simulink model "MMC_phase_hackathon_circuit3_HAAS_20260216"  (R2024b)
settings: Solver=FixedStepDiscrete  StartTime=t_init_sim  StopTime=sim_time  FixedStep=Ts  RelTol=1e-3
values from neighbouring files (symbols this model uses):
  a = 1    [param_phase_circuit3_20260216.m]
  C1low1_active = 1    [script_MMC_phase_circuit3_twist_20260216.m]
  C2low1_active = 1    [script_MMC_phase_circuit3_twist_20260216.m]
  C_bus = 4400e-6    (= 0.0044)    [param_phase_circuit3_20260216.m]
  C_M_extra = C_m-twist_high_side_C    [param_phase_circuit3_20260216.m]
  duty_cycle = 0.95    [script_MMC_phase_circuit3_twist_20260216.m]
  f0 = 50    [param_phase_circuit3_20260216.m]
  feeder_current_lower_rate_limit = -10    [script_MMC_phase_circuit3_twist_20260216.m]    (also in twist_parameters.m = -500)
  feeder_current_tab = [0.328 0.217 0.162 0.132 0.109 0.094 0.083 0.075 0.068 0.062 0.058 0.054 ... (42 elements, 14x3)]    [feeder_current.mat]
  feeder_current_upper_rate_limit = 0.386/(20e-3)    (= 19.3)    [twist_parameters.m]
  is6VExternallySupplied = true    [script_MMC_phase_circuit3_twist_20260216.m]
  isFeederJumperOpen = true    [script_MMC_phase_circuit3_twist_20260216.m]
  L_arm = 60e-3    (= 0.06)    [param_phase_circuit3_20260216.m]
  m = 1    [param_phase_circuit3_20260216.m]
  N = 5    [param_phase_circuit3_20260216.m]
  power_losses = false    [script_MMC_phase_circuit3_twist_20260216.m]
  R = 15    [param_phase_circuit3_20260216.m]
  source_V = 0    [script_MMC_phase_circuit3_twist_20260216.m]
  time_charge = 0.1    [script_MMC_phase_circuit3_twist_20260216.m]
  time_decharge = 0.6    [script_MMC_phase_circuit3_twist_20260216.m]
  Ts = 5e-7    (= 5e-07)    [script_MMC_phase_circuit3_twist_20260216.m]
  twist_data_acquisition_delay = 50e-9    (= 5e-08)    [script_MMC_phase_circuit3_twist_20260216.m]    (also in twist_parameters.m)
  twist_data_sampling_period = 1/twist_freq_data_sampling    (= 5e-05)    [script_MMC_phase_circuit3_twist_20260216.m]    (also in twist_parameters.m)
  twist_dead_time = 200e-9    (= 2e-07)    [twist_parameters.m]
  twist_freq_switching = 200e3    (= 200000)    [twist_parameters.m]
  twist_high_side_adc_R = 1/(1/2e6 + 1/2e6 + 1/(330e3+5.6e3))    (= 251272.836178)    [twist_parameters.m]
  twist_high_side_C = 33e-6*4 + 4.7e-6*12    (= 0.0001884)    [twist_parameters.m]
  twist_high_side_feeder_R = 47e3+4.7e3    (= 51700)    [twist_parameters.m]
  twist_high_side_rC = 0.1    [twist_parameters.m]
  twist_low_side_adc_R = 150e3+470    (= 150470)    [twist_parameters.m]
  twist_low_side_C_ceramic = 3*4.7e-6    (= 1.41e-05)    [twist_parameters.m]
  twist_low_side_C_electrolytic = 47e-6    (= 4.7e-05)    [twist_parameters.m]
  twist_low_side_L = 33e-6    (= 3.3e-05)    [twist_parameters.m]
  twist_low_side_rC = 700e-3    (= 0.7)    [twist_parameters.m]
  twist_low_side_rL = 20e-3    (= 0.02)    [twist_parameters.m]
  twist_R_VCC = (tau_VCC/twist_high_side_C  - twist_high_side_rC)/(1-(tau_VCC/twist_high_side_C - twist_high_side_rC)/R_parallel)    (= 1110.74997822)    [twist_parameters.m]
  VDC = 48    [param_phase_circuit3_20260216.m]
undefined symbols (not defined in the file or in its folder): C_SM, feeder_current, gcbh, sps_rtmsupport, twist_low_side_lC
libraries: spsSeriesRLCBranchLib x133, spsTriangleGeneratorLib x60, spsMosfetLib x60, spsVoltageMeasurementLib x55, spsCurrentMeasurementLib x43, spsControlledCurrentSourceLib x30, spsDiodeLib x22, spsIdealSwitchLib x20, spsControlledVoltageSourceLib x1, spsGroundLib x1, spsMeanLib x1, spspowerguiLib x1
(part 5 of 18)

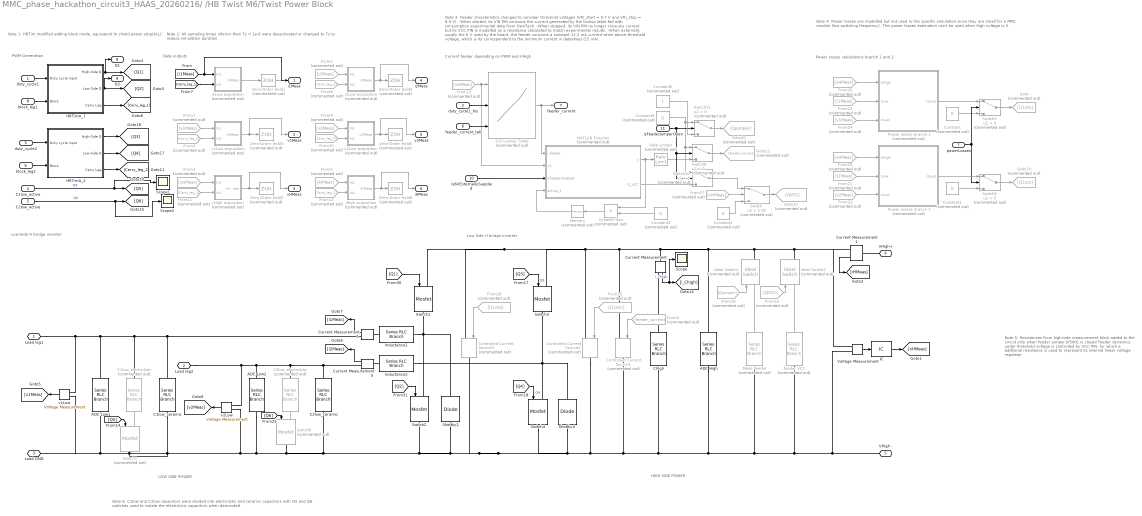
== system MMC_phase_hackathon_circuit3_HAAS_20260216/ /HB Twist M6/Twist Power Block ==
  note: Power losses calculations branch 1 and 2
  note: Current feeder depending on PWM and VHigh
  note: LOW SIDE POWER
  note: Data outputs
  note: PWM Generation
  note: Low-Side H bridge inverter
  note: Low Side H bridge inverter
  note: HIGH SIDE POWER
  note: Note 1:
      | HRTim modified adding block mode, equivalent to shield.power.stop(ALL);
  note: Note 2:
      | All sampling times inferior than Ts = 1e-6 were desactivated or changed to Ts to reduce simulation duration
  note: Note 3:
      | Feeder chracteristics changed to consider threshold voltages (Vth_start = 9.7 V and Vth_stop = 8.9 V).
      | -When started, its VIN PIN consums the current generated by the lookup table fed with consumption experimental data from OwnTech.
      | -When stopped, its VIN PIN no longer consums current but its VCC PIN is modelled as a resistance calculated to match experimental results.
      | -When externally supply the 6 V used by the board, the feeder consums a constant 11.2 mA current when above threshold voltage, which is its correspondent to the minimum current in datasheet (15 mA).
  note: Note 5:
      |
      | Resistances from high-side measurement block added to the circuit only when feeder jumper JP5001 is closed
      |
      | Feeder dynamics under threshold voltage is controlled by VCC PIN, for which a addtional resistance is used to represent its internal linear voltage regulator
  note: Note 4:
      | Power losses are modelled but not used in this specific simulation since they are small for a MMC module (low switching frequency).
      |
      | This power losses estimation can't be used when High voltage is 0.
  note: Note 6:
      | C1low and C2low capacitors were divided into electrolytic and ceramic capacitors with Q5 and Q6 switches used to isolate the electrolytic capacitors when demanded.
  duty_cycle1 : Inport
  duty_cycle1_bis : Inport  Port=2
  duty_cycle2 : Inport  Port=3
  C1low_active : Inport  Port=4
  C2low_active : Inport  Port=5
  feeder_current_tab : Inport  Port=6
  powerLosses : Inport  Port=7
  block_leg1 : Inport  Port=8
  block_leg2 : Inport  Port=9
  is6VExternallySupplied : Inport  Port=10
  isFeederJumperOpen : Inport  Port=11
  2-D Lookup Table : Lookup_n-D  Commented=on  LookupTableObject=feeder_current_tab  BreakpointsSpecification=Even spacing  BreakpointsForDimension1=[1:4]  BreakpointsForDimension2=[1:3]  BreakpointsForDimension1FirstPoint=feeder_VHigh_min  BreakpointsForDimension2FirstPoint=feeder_duty_min  BreakpointsForDimension1Spacing=feeder_VHigh_spacing  BreakpointsForDimension2Spacing=feeder_duty_spacing  TableSource=Input port  Table=feeder_current  InternalRulePriority=Speed  RndMeth=Simplest
      settings: InputPortMap=u0,u1,p221
  ADC High : spsSeriesRLCBranchLib/Series RLC Branch  LConnTagsString=__new0  RConnTagsString=__new0  BranchType=R  Resistance=twist_high_side_adc_R  Inductance=twist_low_side_L  SetiL0=off  InitialCurrent=0  Capacitance=1e-6  Setx0=off  InitialVoltage=0  Measurements=None
  ADC Low1 : spsSeriesRLCBranchLib/Series RLC Branch  LConnTagsString=__new0  RConnTagsString=__new0  BranchType=R  Resistance=twist_low_side_adc_R  Inductance=twist_low_side_L  SetiL0=off  InitialCurrent=0  Capacitance=1e-6  Setx0=off  InitialVoltage=0  Measurements=Branch voltage
  ADC Low2 : spsSeriesRLCBranchLib/Series RLC Branch  LConnTagsString=__new0  RConnTagsString=__new0  BranchType=R  Resistance=twist_low_side_adc_R  Inductance=twist_low_side_L  SetiL0=off  InitialCurrent=0  Capacitance=1e-6  Setx0=off  InitialVoltage=0  Measurements=Branch voltage
  C1low_ceramic : spsSeriesRLCBranchLib/Series RLC Branch  LConnTagsString=__new0  RConnTagsString=__new0  BranchType=C  Resistance=twist_low_side_rC  Inductance=1e-3  SetiL0=off  InitialCurrent=0  Capacitance=twist_low_side_C_ceramic  Setx0=off  InitialVoltage=source_V  Measurements=None
  C1low_electrolytic : spsSeriesRLCBranchLib/Series RLC Branch  Commented=on  LConnTagsString=__new0  RConnTagsString=__new0  BranchType=RC  Resistance=twist_low_side_rC  Inductance=twist_low_side_lC  SetiL0=off  InitialCurrent=0  Capacitance=twist_low_side_C_electrolytic  Setx0=off  InitialVoltage=source_V  Measurements=None
  C2low_ceramic : spsSeriesRLCBranchLib/Series RLC Branch  LConnTagsString=__new0  RConnTagsString=__new0  BranchType=C  Resistance=twist_low_side_rC  Inductance=1e-3  SetiL0=off  InitialCurrent=0  Capacitance=twist_low_side_C_ceramic  Setx0=off  InitialVoltage=source_V  Measurements=None
  C2low_electrolytic : spsSeriesRLCBranchLib/Series RLC Branch  Commented=on  LConnTagsString=__new0  RConnTagsString=__new0  BranchType=RC  Resistance=twist_low_side_rC  Inductance=twist_low_side_lC  SetiL0=off  InitialCurrent=0  Capacitance=twist_low_side_C_electrolytic  Setx0=off  InitialVoltage=source_V  Measurements=None
  Chigh : spsSeriesRLCBranchLib/Series RLC Branch  LConnTagsString=__new0  RConnTagsString=__new0  BranchType=RC  Resistance=twist_high_side_rC  Inductance=1e-3  SetiL0=off  InitialCurrent=0  Capacitance=twist_high_side_C  Setx0=on  InitialVoltage=source_V  Measurements=None
  Constant{,1..2,4,6} (5 alike) : Constant  Commented=on  Value=0
  Constant5 : Constant  Commented=on
  Controlled Current Source1 : spsControlledCurrentSourceLib/Controlled Current Source  Commented=on  Initialize=on  Source_Type=AC  Amplitude=0  Phase=0  Frequency=0  Measurements=None
  Controlled Current Source2 : spsControlledCurrentSourceLib/Controlled Current Source  Commented=on  Initialize=on  Source_Type=AC  Amplitude=0  Phase=0  Frequency=0  Measurements=None
  Controlled Current Source3 : spsControlledCurrentSourceLib/Controlled Current Source  Commented=on  Initialize=on  Source_Type=AC  Amplitude=0  Phase=0  Frequency=0  Measurements=None
  Current Measurement{,1,5..6} (4 alike) : spsCurrentMeasurementLib/Current Measurement  PhasorSimulation=off  OutputType=Complex  PSBequivalent=0
  From1 : From  Commented=on  GotoTag=v1Meas
  From10 : From  Commented=on  GotoTag=Carry_leg_2
  From11 : From  Commented=on  GotoTag=Carry_leg_1
  From12 : From  Commented=on  GotoTag=Carry_leg_2
  From{3,13,19..20,27} (5 alike) : From  Commented=on  GotoTag=vHMeas
  From15 : From  Commented=on  GotoTag=QVCC
  From16 : From  Commented=on  GotoTag=i2Loss
  From2 : From  Commented=on  GotoTag=i2Meas
  From21 : From  Commented=on  GotoTag=i2Meas
  From22 : From  Commented=on  GotoTag=v2Meas
  From23 : From  Commented=on  GotoTag=i1Meas
  From24 : From  Commented=on  GotoTag=v1Meas
  From26 : From  Commented=on  GotoTag=Qjumper
  From28 : From  Commented=on  GotoTag=i1Loss
  From4 : From  Commented=on  GotoTag=v2Meas
  From5 : From  Commented=on  GotoTag=iHMeas
  From6 : From  Commented=on  GotoTag=feeder_current
  From8 : From  Commented=on  GotoTag=Carry_leg_2
  From9 : From  Commented=on  GotoTag=Carry_leg_1
  Goto : Goto  Commented=on  GotoTag=i1Loss
  Goto12 : Goto  Commented=on  GotoTag=feeder_current
  Goto13 : Goto  Commented=on  GotoTag=QVCC
  Goto19 : Goto  Commented=on  GotoTag=i2Loss
  Goto20 : Goto  Commented=on  GotoTag=Qjumper
  GreaterThan : RelationalOperator  Commented=on  Operator=>  OutDataTypeStr=boolean  RndMeth=Simplest  InputSameDT=off
  HRTimA_1 : Subsystem
  HRTimA_2 : Subsystem
  IC : InitialCondition  Value=source_V
  Ideal Switch1 : spsIdealSwitchLib/Ideal Switch  Commented=on  Ron=0.001  Lon=0  IC=0  Rs=1e5  Cs=inf  Measurements=on
  Ideal Switch2 : spsIdealSwitchLib/Ideal Switch  Commented=on  Ron=0.001  Lon=0  IC=0  Rs=1e5  Cs=inf  Measurements=on
  Inductance1 : spsSeriesRLCBranchLib/Series RLC Branch  LConnTagsString=__new0  RConnTagsString=__new0  BranchType=RL  Resistance=twist_low_side_rL  Inductance=twist_low_side_L  SetiL0=off  InitialCurrent=0  Capacitance=1e-6  Setx0=off  InitialVoltage=0  Measurements=None
  Inductance2 : spsSeriesRLCBranchLib/Series RLC Branch  LConnTagsString=__new0  RConnTagsString=__new0  BranchType=RL  Resistance=twist_low_side_rL  Inductance=twist_low_side_L  SetiL0=off  InitialCurrent=0  Capacitance=1e-6  Setx0=off  InitialVoltage=0  Measurements=None
  MATLAB Function : MATLAB Function  Commented=on  TreatAsAtomicUnit=on
  Meas Feeder : spsSeriesRLCBranchLib/Series RLC Branch  Commented=on  LConnTagsString=__new0  RConnTagsString=__new0  BranchType=R  Resistance=twist_high_side_feeder_R  Inductance=twist_low_side_L  SetiL0=off  InitialCurrent=0  Capacitance=1e-6  Setx0=off  InitialVoltage=0  Measurements=None
  Memory : Memory  Commented=on  InheritSampleTime=on  LinearizeAsDelay=on
  Power losses branch 1 : Subsystem  Commented=on
  Power losses branch 2 : Subsystem  Commented=on
  Rate Limiter : RateLimiter  Commented=on  RisingSlewLimit=feeder_current_upper_rate_limit  FallingSlewLimit=feeder_current_lower_rate_limit  SampleTimeMode=inherited
  Scope : Scope
  Scope1 : Scope
  Scope2 : Scope
  Shottky2 : spsDiodeLib/Diode  Ron=twist_shottky_Ron  Lon=0  Vf=twist_shottky_Vf  IC=0  UseSnubber=0  Rs=twist_shottky_Rs  Cs=twist_shottky_Cs  Measurements=off
  Shottky4 : spsDiodeLib/Diode  Ron=twist_shottky_Ron  Lon=0  Vf=twist_shottky_Vf  IC=0  UseSnubber=0  Rs=twist_shottky_Rs  Cs=twist_shottky_Cs  Measurements=off
  Switch : Switch  Commented=on  Criteria=u2 > Threshold  Threshold=2.05  SaturateOnIntegerOverflow=off  InputSameDT=off
  Switch{1..4} (4 alike) : spsMosfetLib/Mosfet  Ron=twist_FET_Ron  Lon=0  Rd=twist_FET_Rd  Vfd=twist_FET_Vf  IC=0  Rs=twist_FET_Rs  Cs=twist_FET_Cs  Measurements=off
  Switch{5..6,9..11} (5 alike) : Switch  Commented=on  Criteria=u2 > Threshold  SaturateOnIntegerOverflow=off  InputSameDT=off
  Switch7 : spsMosfetLib/Mosfet  Commented=on  Ron=twist_FET_Clow_Ron  Lon=0  Rd=twist_FET_Clow_Ron  Vfd=0  IC=0  Rs=twist_FET_Rs  Cs=twist_FET_Cs  Measurements=off
  Switch8 : spsMosfetLib/Mosfet  Commented=on  Ron=twist_FET_Clow_Ron  Lon=0  Rd=twist_FET_Clow_Ron  Vfd=0  IC=0  Rs=twist_FET_Rs  Cs=twist_FET_Cs  Measurements=off
  Voltage Measurement : spsVoltageMeasurementLib/Voltage Measurement  PhasorSimulation=off  OutputType=Complex  PSBequivalent=0
  Zero-Order Hold{1..6} (6 alike) : ZeroOrderHold  Commented=on  SampleTime=twist_data_sampling_period
  feeder VCC : spsSeriesRLCBranchLib/Series RLC Branch  Commented=on  LConnTagsString=__new0  RConnTagsString=__new0  BranchType=R  Resistance=twist_R_VCC  Inductance=twist_low_side_L  SetiL0=off  InitialCurrent=0  Capacitance=1e-6  Setx0=off  InitialVoltage=0  Measurements=None
  i1Low acquisition : Subsystem  Commented=on
  i2Low acquisition : Subsystem  Commented=on
  iHigh acquisition : Subsystem  Commented=on
  v1Low : spsVoltageMeasurementLib/Voltage Measurement  PhasorSimulation=off  OutputType=Complex  PSBequivalent=0
  v1Low acquisition : Subsystem  Commented=on
  v2Low : spsVoltageMeasurementLib/Voltage Measurement  PhasorSimulation=off  OutputType=Complex  PSBequivalent=0
  v2Low acquisition : Subsystem  Commented=on
  vHigh acquisition : Subsystem  Commented=on
  Load leg1 : PMIOPort  Side=Left
  Load leg2 : PMIOPort  Port=2  Side=Left
  Load GND : PMIOPort  Port=3  Side=Left
  VHigh+ : PMIOPort  Port=4  Side=Right
  VHigh - : PMIOPort  Port=5  Side=Right
  i1Meas : Outport
  v1Meas : Outport  Port=2
  vHMeas : Outport  Port=3
  i2Meas : Outport  Port=4
  v2Meas : Outport  Port=5
  iHMeas : Outport  Port=6
  feeder_current : Outport  Port=7
  Q1 : Outport  Port=8
  Q2 : Outport  Port=9
  wires:
  duty_cycle1/1 -> HRTimA_1/1(Duty cycle input)
  HRTimA_1/2(Low-Side Q) -> [Q2], Q2/1
  From1/1 -> v1Low acquisition/1(In1)
  C1low_active/1 -> Scope1/1, [Q5]  "Q5"
  HRTimA_1/1(High-Side Q) -> [Q1], Q1/1
  HRTimA_2/1(High-Side Q) -> [Q3]
  HRTimA_2/2(Low-Side Q) -> [Q4]
  From11/1 -> vHigh acquisition/2(In2)
  From3/1 -> vHigh acquisition/1(In1)
  From2/1 -> i2Low acquisition/1(In1)
  From8/1 -> i2Low acquisition/2(In2)
  From4/1 -> v2Low acquisition/1(In1)
  From10/1 -> v2Low acquisition/2(In2)
  From5/1 -> iHigh acquisition/1(In1)
  From12/1 -> iHigh acquisition/2(In2)
  From9/1 -> v1Low acquisition/2(In2)
  v1Low acquisition/1(v1Meas) -> v1Meas/1, Zero-Order Hold3/1
  i2Low acquisition/1(i2Meas) -> i2Meas/1, Zero-Order Hold4/1
  v2Low acquisition/1(v2Meas) -> v2Meas/1, Zero-Order Hold5/1
  iHigh acquisition/1(iHMeas) -> iHMeas/1, Zero-Order Hold6/1
  vHigh acquisition/1(vHMeas) -> vHMeas/1, Zero-Order Hold2/1
  HRTimA_2/3(Carry Leg) -> [Carry_leg_2]
  HRTimA_1/3(Carry Leg) -> [Carry_leg_1]
  duty_cycle2/1 -> HRTimA_2/1(Duty cycle input)
  From13/1 -> MATLAB Function/2(vC), 2-D Lookup Table/1
  v2Low/1 -> [v2Meas]
  [Q3] -> Switch3/1  "Q3"
  Current Measurement6/1 -> [i1Meas]
  [Q1] -> Switch1/1
  [Q4] -> Switch4/1  "Q4"
  v1Low/1 -> [v1Meas]
  [Q2] -> Switch2/1
  Current Measurement1/1 -> [iHMeas]
  Current Measurement5/1 -> [i2Meas]
  [Carry_leg_1] -> i1Low acquisition/2(In2)
  [i1Meas] -> i1Meas/1, i1Low acquisition/1(In1)
  i1Low acquisition/1(i1Meas) -> Zero-Order Hold1/1
  Voltage Measurement/1 -> IC/1
  IC/1 -> [vHMeas]
  From20/1 -> Power losses branch 1/1(VHigh)
  From23/1 -> Power losses branch 1/2(ILow)
  From24/1 -> Power losses branch 1/3(VLow)
  Power losses branch 1/1(i1Loss) -> Switch5/1
  Switch5/1 -> Goto/1
  Constant/1 -> Switch5/3
  feeder_current_tab/1 -> 2-D Lookup Table/3
  duty_cycle1_bis/1 -> 2-D Lookup Table/2
  [Q5] -> Switch7/1
  C2low_active/1 -> Scope2/1, [Q6]  "Q6"
  From6/1 -> Controlled Current Source1/1
  block_leg1/1 -> HRTimA_1/2(Block)
  Current Measurement/1 -> Scope/1, [i_Chigh]  "i_Chigh"
  block_leg2/1 -> HRTimA_2/2(Block)
  GreaterThan/1 -> Memory/1
  Constant2/1 -> GreaterThan/2
  From15/1 -> Ideal Switch2/1
  2-D Lookup Table/1 -> feeder_current/1, MATLAB Function/1(i_feeder)
  MATLAB Function/1(y) -> GreaterThan/1, Rate Limiter/1
  powerLosses/1 -> Switch5/2, Switch6/2
  From19/1 -> Power losses branch 2/1(VHigh)
  From21/1 -> Power losses branch 2/2(ILow)
  From22/1 -> Power losses branch 2/3(VLow)
  Switch6/1 -> Goto19/1
  Constant1/1 -> Switch6/3
  Power losses branch 2/1(i1Loss) -> Switch6/1
  is6VExternallySupplied/1 -> MATLAB Function/3(isfeederdisabled)
  Memory/1 -> MATLAB Function/4(active_1)
  From27/1 -> Switch/2
  Constant4/1 -> Switch/3
  [Q6] -> Switch8/1
  Switch9/1 -> Goto12/1
  Rate Limiter/1 -> Switch9/3
  MATLAB Function/2(Q_VCC) -> Switch10/3
  Constant6/1 -> Switch11/1, Switch10/1, Switch9/1
  isFeederJumperOpen/1 -> Switch11/2, Switch9/2, Switch10/2
  Switch/1 -> Goto13/1
  Switch10/1 -> Switch/1
  Constant5/1 -> Switch11/3
  Switch11/1 -> Goto20/1
  From26/1 -> Ideal Switch1/1
  From16/1 -> Controlled Current Source2/1
  From28/1 -> Controlled Current Source3/1
  Zero-Order Hold1/1 -> ?
  connections:
  Inductance2/LConn1 -- Current Measurement5/LConn1
  Current Measurement6/LConn1 -- Inductance1/LConn1
  VHigh+/RConn1 -- Current Measurement1/LConn1
  v2Low/LConn1 -- Load leg2/RConn1 -- ADC Low2/LConn1 -- C2low_electrolytic/LConn1 -- C2low_ceramic/LConn1 -- Current Measurement5/RConn1
  Switch4/LConn1 -- Switch3/RConn1 -- Shottky4/RConn1 -- Inductance2/RConn1
  v1Low/LConn1 -- Load leg1/RConn1 -- C1low_ceramic/LConn1 -- Current Measurement6/RConn1 -- C1low_electrolytic/LConn1 -- ADC Low1/LConn1
  Current Measurement/RConn1 -- Chigh/LConn1
  ADC High/RConn1 -- Meas Feeder/RConn1 -- feeder VCC/RConn1 -- Voltage Measurement/LConn2 -- VHigh -/RConn1 -- Chigh/RConn1 -- Controlled Current Source2/RConn1 -- Controlled Current Source3/RConn1 -- Switch2/RConn1 -- Load GND/RConn1 -- v1Low/LConn2 -- ADC Low1/RConn1 -- Switch7/RConn1 -- C1low_ceramic/RConn1 -- v2Low/LConn2 -- ADC Low2/RConn1 -- Switch8/RConn1 -- C2low_ceramic/RConn1 -- Shottky2/LConn1 -- Switch4/RConn1 -- Shottky4/LConn1 -- Controlled Current Source1/RConn1
  Switch7/LConn1 -- C1low_electrolytic/RConn1
  Switch8/LConn1 -- C2low_electrolytic/RConn1
  Inductance1/RConn1 -- Shottky2/RConn1 -- Switch2/LConn1 -- Switch1/RConn1
  Ideal Switch2/LConn1 -- feeder VCC/LConn1
  Current Measurement/LConn1 -- Ideal Switch1/RConn1 -- Voltage Measurement/LConn1 -- Current Measurement1/RConn1 -- Ideal Switch2/RConn1 -- ADC High/LConn1 -- Controlled Current Source2/LConn1 -- Controlled Current Source3/LConn1 -- Switch1/LConn1 -- Switch3/LConn1 -- Controlled Current Source1/LConn1
  Meas Feeder/LConn1 -- Ideal Switch1/LConn1

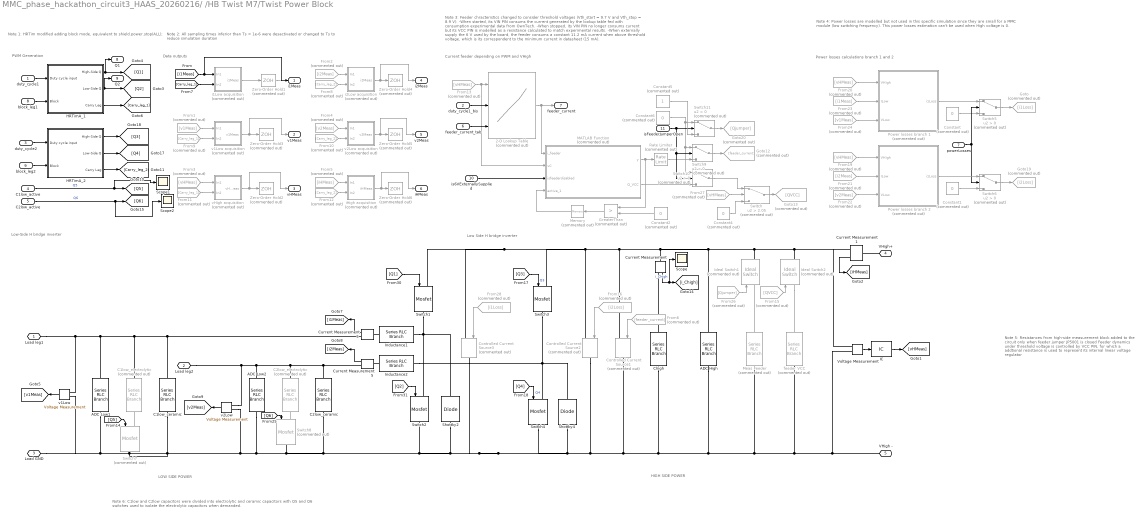
== system MMC_phase_hackathon_circuit3_HAAS_20260216/ /HB Twist M7/Twist Power Block ==
  note: Power losses calculations branch 1 and 2
  note: Current feeder depending on PWM and VHigh
  note: LOW SIDE POWER
  note: Data outputs
  note: PWM Generation
  note: Low-Side H bridge inverter
  note: Low Side H bridge inverter
  note: HIGH SIDE POWER
  note: Note 1:
      | HRTim modified adding block mode, equivalent to shield.power.stop(ALL);
  note: Note 2:
      | All sampling times inferior than Ts = 1e-6 were desactivated or changed to Ts to reduce simulation duration
  note: Note 3:
      | Feeder chracteristics changed to consider threshold voltages (Vth_start = 9.7 V and Vth_stop = 8.9 V).
      | -When started, its VIN PIN consums the current generated by the lookup table fed with consumption experimental data from OwnTech.
      | -When stopped, its VIN PIN no longer consums current but its VCC PIN is modelled as a resistance calculated to match experimental results.
      | -When externally supply the 6 V used by the board, the feeder consums a constant 11.2 mA current when above threshold voltage, which is its correspondent to the minimum current in datasheet (15 mA).
  note: Note 5:
      |
      | Resistances from high-side measurement block added to the circuit only when feeder jumper JP5001 is closed
      |
      | Feeder dynamics under threshold voltage is controlled by VCC PIN, for which a addtional resistance is used to represent its internal linear voltage regulator
  note: Note 4:
      | Power losses are modelled but not used in this specific simulation since they are small for a MMC module (low switching frequency).
      |
      | This power losses estimation can't be used when High voltage is 0.
  note: Note 6:
      | C1low and C2low capacitors were divided into electrolytic and ceramic capacitors with Q5 and Q6 switches used to isolate the electrolytic capacitors when demanded.
  duty_cycle1 : Inport
  duty_cycle1_bis : Inport  Port=2
  duty_cycle2 : Inport  Port=3
  C1low_active : Inport  Port=4
  C2low_active : Inport  Port=5
  feeder_current_tab : Inport  Port=6
  powerLosses : Inport  Port=7
  block_leg1 : Inport  Port=8
  block_leg2 : Inport  Port=9
  is6VExternallySupplied : Inport  Port=10
  isFeederJumperOpen : Inport  Port=11
  2-D Lookup Table : Lookup_n-D  Commented=on  LookupTableObject=feeder_current_tab  BreakpointsSpecification=Even spacing  BreakpointsForDimension1=[1:4]  BreakpointsForDimension2=[1:3]  BreakpointsForDimension1FirstPoint=feeder_VHigh_min  BreakpointsForDimension2FirstPoint=feeder_duty_min  BreakpointsForDimension1Spacing=feeder_VHigh_spacing  BreakpointsForDimension2Spacing=feeder_duty_spacing  TableSource=Input port  Table=feeder_current  InternalRulePriority=Speed  RndMeth=Simplest
      settings: InputPortMap=u0,u1,p221
  ADC High : spsSeriesRLCBranchLib/Series RLC Branch  LConnTagsString=__new0  RConnTagsString=__new0  BranchType=R  Resistance=twist_high_side_adc_R  Inductance=twist_low_side_L  SetiL0=off  InitialCurrent=0  Capacitance=1e-6  Setx0=off  InitialVoltage=0  Measurements=None
  ADC Low1 : spsSeriesRLCBranchLib/Series RLC Branch  LConnTagsString=__new0  RConnTagsString=__new0  BranchType=R  Resistance=twist_low_side_adc_R  Inductance=twist_low_side_L  SetiL0=off  InitialCurrent=0  Capacitance=1e-6  Setx0=off  InitialVoltage=0  Measurements=Branch voltage
  ADC Low2 : spsSeriesRLCBranchLib/Series RLC Branch  LConnTagsString=__new0  RConnTagsString=__new0  BranchType=R  Resistance=twist_low_side_adc_R  Inductance=twist_low_side_L  SetiL0=off  InitialCurrent=0  Capacitance=1e-6  Setx0=off  InitialVoltage=0  Measurements=Branch voltage
  C1low_ceramic : spsSeriesRLCBranchLib/Series RLC Branch  LConnTagsString=__new0  RConnTagsString=__new0  BranchType=C  Resistance=twist_low_side_rC  Inductance=1e-3  SetiL0=off  InitialCurrent=0  Capacitance=twist_low_side_C_ceramic  Setx0=off  InitialVoltage=source_V  Measurements=None
  C1low_electrolytic : spsSeriesRLCBranchLib/Series RLC Branch  Commented=on  LConnTagsString=__new0  RConnTagsString=__new0  BranchType=RC  Resistance=twist_low_side_rC  Inductance=twist_low_side_lC  SetiL0=off  InitialCurrent=0  Capacitance=twist_low_side_C_electrolytic  Setx0=off  InitialVoltage=source_V  Measurements=None
  C2low_ceramic : spsSeriesRLCBranchLib/Series RLC Branch  LConnTagsString=__new0  RConnTagsString=__new0  BranchType=C  Resistance=twist_low_side_rC  Inductance=1e-3  SetiL0=off  InitialCurrent=0  Capacitance=twist_low_side_C_ceramic  Setx0=off  InitialVoltage=source_V  Measurements=None
  C2low_electrolytic : spsSeriesRLCBranchLib/Series RLC Branch  Commented=on  LConnTagsString=__new0  RConnTagsString=__new0  BranchType=RC  Resistance=twist_low_side_rC  Inductance=twist_low_side_lC  SetiL0=off  InitialCurrent=0  Capacitance=twist_low_side_C_electrolytic  Setx0=off  InitialVoltage=source_V  Measurements=None
  Chigh : spsSeriesRLCBranchLib/Series RLC Branch  LConnTagsString=__new0  RConnTagsString=__new0  BranchType=RC  Resistance=twist_high_side_rC  Inductance=1e-3  SetiL0=off  InitialCurrent=0  Capacitance=twist_high_side_C  Setx0=on  InitialVoltage=source_V  Measurements=None
  Constant{,1..2,4,6} (5 alike) : Constant  Commented=on  Value=0
  Constant5 : Constant  Commented=on
  Controlled Current Source1 : spsControlledCurrentSourceLib/Controlled Current Source  Commented=on  Initialize=on  Source_Type=AC  Amplitude=0  Phase=0  Frequency=0  Measurements=None
  Controlled Current Source2 : spsControlledCurrentSourceLib/Controlled Current Source  Commented=on  Initialize=on  Source_Type=AC  Amplitude=0  Phase=0  Frequency=0  Measurements=None
  Controlled Current Source3 : spsControlledCurrentSourceLib/Controlled Current Source  Commented=on  Initialize=on  Source_Type=AC  Amplitude=0  Phase=0  Frequency=0  Measurements=None
  Current Measurement{,1,5..6} (4 alike) : spsCurrentMeasurementLib/Current Measurement  PhasorSimulation=off  OutputType=Complex  PSBequivalent=0
  From1 : From  Commented=on  GotoTag=v1Meas
  From10 : From  Commented=on  GotoTag=Carry_leg_2
  From11 : From  Commented=on  GotoTag=Carry_leg_1
  From12 : From  Commented=on  GotoTag=Carry_leg_2
  From{3,13,19..20,27} (5 alike) : From  Commented=on  GotoTag=vHMeas
  From15 : From  Commented=on  GotoTag=QVCC
  From16 : From  Commented=on  GotoTag=i2Loss
  From2 : From  Commented=on  GotoTag=i2Meas
  From21 : From  Commented=on  GotoTag=i2Meas
  From22 : From  Commented=on  GotoTag=v2Meas
  From23 : From  Commented=on  GotoTag=i1Meas
  From24 : From  Commented=on  GotoTag=v1Meas
  From26 : From  Commented=on  GotoTag=Qjumper
  From28 : From  Commented=on  GotoTag=i1Loss
  From4 : From  Commented=on  GotoTag=v2Meas
  From5 : From  Commented=on  GotoTag=iHMeas
  From6 : From  Commented=on  GotoTag=feeder_current
  From8 : From  Commented=on  GotoTag=Carry_leg_2
  From9 : From  Commented=on  GotoTag=Carry_leg_1
  Goto : Goto  Commented=on  GotoTag=i1Loss
  Goto12 : Goto  Commented=on  GotoTag=feeder_current
  Goto13 : Goto  Commented=on  GotoTag=QVCC
  Goto19 : Goto  Commented=on  GotoTag=i2Loss
  Goto20 : Goto  Commented=on  GotoTag=Qjumper
  GreaterThan : RelationalOperator  Commented=on  Operator=>  OutDataTypeStr=boolean  RndMeth=Simplest  InputSameDT=off
  HRTimA_1 : Subsystem
  HRTimA_2 : Subsystem
  IC : InitialCondition  Value=source_V
  Ideal Switch1 : spsIdealSwitchLib/Ideal Switch  Commented=on  Ron=0.001  Lon=0  IC=0  Rs=1e5  Cs=inf  Measurements=on
  Ideal Switch2 : spsIdealSwitchLib/Ideal Switch  Commented=on  Ron=0.001  Lon=0  IC=0  Rs=1e5  Cs=inf  Measurements=on
  Inductance1 : spsSeriesRLCBranchLib/Series RLC Branch  LConnTagsString=__new0  RConnTagsString=__new0  BranchType=RL  Resistance=twist_low_side_rL  Inductance=twist_low_side_L  SetiL0=off  InitialCurrent=0  Capacitance=1e-6  Setx0=off  InitialVoltage=0  Measurements=None
  Inductance2 : spsSeriesRLCBranchLib/Series RLC Branch  LConnTagsString=__new0  RConnTagsString=__new0  BranchType=RL  Resistance=twist_low_side_rL  Inductance=twist_low_side_L  SetiL0=off  InitialCurrent=0  Capacitance=1e-6  Setx0=off  InitialVoltage=0  Measurements=None
  MATLAB Function : MATLAB Function  Commented=on  TreatAsAtomicUnit=on
  Meas Feeder : spsSeriesRLCBranchLib/Series RLC Branch  Commented=on  LConnTagsString=__new0  RConnTagsString=__new0  BranchType=R  Resistance=twist_high_side_feeder_R  Inductance=twist_low_side_L  SetiL0=off  InitialCurrent=0  Capacitance=1e-6  Setx0=off  InitialVoltage=0  Measurements=None
  Memory : Memory  Commented=on  InheritSampleTime=on  LinearizeAsDelay=on
  Power losses branch 1 : Subsystem  Commented=on
  Power losses branch 2 : Subsystem  Commented=on
  Rate Limiter : RateLimiter  Commented=on  RisingSlewLimit=feeder_current_upper_rate_limit  FallingSlewLimit=feeder_current_lower_rate_limit  SampleTimeMode=inherited
  Scope : Scope
  Scope1 : Scope
  Scope2 : Scope
  Shottky2 : spsDiodeLib/Diode  Ron=twist_shottky_Ron  Lon=0  Vf=twist_shottky_Vf  IC=0  UseSnubber=0  Rs=twist_shottky_Rs  Cs=twist_shottky_Cs  Measurements=off
  Shottky4 : spsDiodeLib/Diode  Ron=twist_shottky_Ron  Lon=0  Vf=twist_shottky_Vf  IC=0  UseSnubber=0  Rs=twist_shottky_Rs  Cs=twist_shottky_Cs  Measurements=off
  Switch : Switch  Commented=on  Criteria=u2 > Threshold  Threshold=2.05  SaturateOnIntegerOverflow=off  InputSameDT=off
  Switch{1..4} (4 alike) : spsMosfetLib/Mosfet  Ron=twist_FET_Ron  Lon=0  Rd=twist_FET_Rd  Vfd=twist_FET_Vf  IC=0  Rs=twist_FET_Rs  Cs=twist_FET_Cs  Measurements=off
  Switch{5..6,9..11} (5 alike) : Switch  Commented=on  Criteria=u2 > Threshold  SaturateOnIntegerOverflow=off  InputSameDT=off
  Switch7 : spsMosfetLib/Mosfet  Commented=on  Ron=twist_FET_Clow_Ron  Lon=0  Rd=twist_FET_Clow_Ron  Vfd=0  IC=0  Rs=twist_FET_Rs  Cs=twist_FET_Cs  Measurements=off
  Switch8 : spsMosfetLib/Mosfet  Commented=on  Ron=twist_FET_Clow_Ron  Lon=0  Rd=twist_FET_Clow_Ron  Vfd=0  IC=0  Rs=twist_FET_Rs  Cs=twist_FET_Cs  Measurements=off
  Voltage Measurement : spsVoltageMeasurementLib/Voltage Measurement  PhasorSimulation=off  OutputType=Complex  PSBequivalent=0
  Zero-Order Hold{1..6} (6 alike) : ZeroOrderHold  Commented=on  SampleTime=twist_data_sampling_period
  feeder VCC : spsSeriesRLCBranchLib/Series RLC Branch  Commented=on  LConnTagsString=__new0  RConnTagsString=__new0  BranchType=R  Resistance=twist_R_VCC  Inductance=twist_low_side_L  SetiL0=off  InitialCurrent=0  Capacitance=1e-6  Setx0=off  InitialVoltage=0  Measurements=None
  i1Low acquisition : Subsystem  Commented=on
  i2Low acquisition : Subsystem  Commented=on
  iHigh acquisition : Subsystem  Commented=on
  v1Low : spsVoltageMeasurementLib/Voltage Measurement  PhasorSimulation=off  OutputType=Complex  PSBequivalent=0
  v1Low acquisition : Subsystem  Commented=on
  v2Low : spsVoltageMeasurementLib/Voltage Measurement  PhasorSimulation=off  OutputType=Complex  PSBequivalent=0
  v2Low acquisition : Subsystem  Commented=on
  vHigh acquisition : Subsystem  Commented=on
  Load leg1 : PMIOPort  Side=Left
  Load leg2 : PMIOPort  Port=2  Side=Left
  Load GND : PMIOPort  Port=3  Side=Left
  VHigh+ : PMIOPort  Port=4  Side=Right
  VHigh - : PMIOPort  Port=5  Side=Right
  i1Meas : Outport
  v1Meas : Outport  Port=2
  vHMeas : Outport  Port=3
  i2Meas : Outport  Port=4
  v2Meas : Outport  Port=5
  iHMeas : Outport  Port=6
  feeder_current : Outport  Port=7
  Q1 : Outport  Port=8
  Q2 : Outport  Port=9
  wires:
  duty_cycle1/1 -> HRTimA_1/1(Duty cycle input)
  HRTimA_1/2(Low-Side Q) -> [Q2], Q2/1
  From1/1 -> v1Low acquisition/1(In1)
  C1low_active/1 -> Scope1/1, [Q5]  "Q5"
  HRTimA_1/1(High-Side Q) -> [Q1], Q1/1
  HRTimA_2/1(High-Side Q) -> [Q3]
  HRTimA_2/2(Low-Side Q) -> [Q4]
  From11/1 -> vHigh acquisition/2(In2)
  From3/1 -> vHigh acquisition/1(In1)
  From2/1 -> i2Low acquisition/1(In1)
  From8/1 -> i2Low acquisition/2(In2)
  From4/1 -> v2Low acquisition/1(In1)
  From10/1 -> v2Low acquisition/2(In2)
  From5/1 -> iHigh acquisition/1(In1)
  From12/1 -> iHigh acquisition/2(In2)
  From9/1 -> v1Low acquisition/2(In2)
  v1Low acquisition/1(v1Meas) -> v1Meas/1, Zero-Order Hold3/1
  i2Low acquisition/1(i2Meas) -> i2Meas/1, Zero-Order Hold4/1
  v2Low acquisition/1(v2Meas) -> v2Meas/1, Zero-Order Hold5/1
  iHigh acquisition/1(iHMeas) -> iHMeas/1, Zero-Order Hold6/1
  vHigh acquisition/1(vHMeas) -> vHMeas/1, Zero-Order Hold2/1
  HRTimA_2/3(Carry Leg) -> [Carry_leg_2]
  HRTimA_1/3(Carry Leg) -> [Carry_leg_1]
  duty_cycle2/1 -> HRTimA_2/1(Duty cycle input)
  From13/1 -> MATLAB Function/2(vC), 2-D Lookup Table/1
  v2Low/1 -> [v2Meas]
  [Q3] -> Switch3/1  "Q3"
  Current Measurement6/1 -> [i1Meas]
  [Q1] -> Switch1/1
  [Q4] -> Switch4/1  "Q4"
  v1Low/1 -> [v1Meas]
  [Q2] -> Switch2/1
  Current Measurement1/1 -> [iHMeas]
  Current Measurement5/1 -> [i2Meas]
  [Carry_leg_1] -> i1Low acquisition/2(In2)
  [i1Meas] -> i1Meas/1, i1Low acquisition/1(In1)
  i1Low acquisition/1(i1Meas) -> Zero-Order Hold1/1
  Voltage Measurement/1 -> IC/1
  IC/1 -> [vHMeas]
  From20/1 -> Power losses branch 1/1(VHigh)
  From23/1 -> Power losses branch 1/2(ILow)
  From24/1 -> Power losses branch 1/3(VLow)
  Power losses branch 1/1(i1Loss) -> Switch5/1
  Switch5/1 -> Goto/1
  Constant/1 -> Switch5/3
  feeder_current_tab/1 -> 2-D Lookup Table/3
  duty_cycle1_bis/1 -> 2-D Lookup Table/2
  [Q5] -> Switch7/1
  C2low_active/1 -> Scope2/1, [Q6]  "Q6"
  From6/1 -> Controlled Current Source1/1
  block_leg1/1 -> HRTimA_1/2(Block)
  Current Measurement/1 -> Scope/1, [i_Chigh]  "i_Chigh"
  block_leg2/1 -> HRTimA_2/2(Block)
  GreaterThan/1 -> Memory/1
  Constant2/1 -> GreaterThan/2
  From15/1 -> Ideal Switch2/1
  2-D Lookup Table/1 -> feeder_current/1, MATLAB Function/1(i_feeder)
  MATLAB Function/1(y) -> GreaterThan/1, Rate Limiter/1
  powerLosses/1 -> Switch5/2, Switch6/2
  From19/1 -> Power losses branch 2/1(VHigh)
  From21/1 -> Power losses branch 2/2(ILow)
  From22/1 -> Power losses branch 2/3(VLow)
  Switch6/1 -> Goto19/1
  Constant1/1 -> Switch6/3
  Power losses branch 2/1(i1Loss) -> Switch6/1
  is6VExternallySupplied/1 -> MATLAB Function/3(isfeederdisabled)
  Memory/1 -> MATLAB Function/4(active_1)
  From27/1 -> Switch/2
  Constant4/1 -> Switch/3
  [Q6] -> Switch8/1
  Switch9/1 -> Goto12/1
  Rate Limiter/1 -> Switch9/3
  MATLAB Function/2(Q_VCC) -> Switch10/3
  Constant6/1 -> Switch11/1, Switch10/1, Switch9/1
  isFeederJumperOpen/1 -> Switch11/2, Switch9/2, Switch10/2
  Switch/1 -> Goto13/1
  Switch10/1 -> Switch/1
  Constant5/1 -> Switch11/3
  Switch11/1 -> Goto20/1
  From26/1 -> Ideal Switch1/1
  From16/1 -> Controlled Current Source2/1
  From28/1 -> Controlled Current Source3/1
  Zero-Order Hold1/1 -> ?
  connections:
  Inductance2/LConn1 -- Current Measurement5/LConn1
  Current Measurement6/LConn1 -- Inductance1/LConn1
  VHigh+/RConn1 -- Current Measurement1/LConn1
  v2Low/LConn1 -- Load leg2/RConn1 -- ADC Low2/LConn1 -- C2low_electrolytic/LConn1 -- C2low_ceramic/LConn1 -- Current Measurement5/RConn1
  Switch4/LConn1 -- Switch3/RConn1 -- Shottky4/RConn1 -- Inductance2/RConn1
  v1Low/LConn1 -- Load leg1/RConn1 -- C1low_ceramic/LConn1 -- Current Measurement6/RConn1 -- C1low_electrolytic/LConn1 -- ADC Low1/LConn1
  Current Measurement/RConn1 -- Chigh/LConn1
  ADC High/RConn1 -- Meas Feeder/RConn1 -- feeder VCC/RConn1 -- Voltage Measurement/LConn2 -- VHigh -/RConn1 -- Chigh/RConn1 -- Controlled Current Source2/RConn1 -- Controlled Current Source3/RConn1 -- Switch2/RConn1 -- Load GND/RConn1 -- v1Low/LConn2 -- ADC Low1/RConn1 -- Switch7/RConn1 -- C1low_ceramic/RConn1 -- v2Low/LConn2 -- ADC Low2/RConn1 -- Switch8/RConn1 -- C2low_ceramic/RConn1 -- Shottky2/LConn1 -- Switch4/RConn1 -- Shottky4/LConn1 -- Controlled Current Source1/RConn1
  Switch7/LConn1 -- C1low_electrolytic/RConn1
  Switch8/LConn1 -- C2low_electrolytic/RConn1
  Inductance1/RConn1 -- Shottky2/RConn1 -- Switch2/LConn1 -- Switch1/RConn1
  Ideal Switch2/LConn1 -- feeder VCC/LConn1
  Current Measurement/LConn1 -- Ideal Switch1/RConn1 -- Voltage Measurement/LConn1 -- Current Measurement1/RConn1 -- Ideal Switch2/RConn1 -- ADC High/LConn1 -- Controlled Current Source2/LConn1 -- Controlled Current Source3/LConn1 -- Switch1/LConn1 -- Switch3/LConn1 -- Controlled Current Source1/LConn1
  Meas Feeder/LConn1 -- Ideal Switch1/LConn1
